simulink model "MOBATSim"  (R2020b)
settings: Solver=FixedStepAuto  StartTime=0.0  StopTime=Sim_t  FixedStep=0.01  MinStep=0.01  RelTol=1e-2
values from neighbouring files (symbols this model uses):
  Vehicles = evalin('base','Vehicles')    [I2V.m]    (also in VehicleSensors.m)
undefined symbols (not defined in the file or in its folder): Sim_Ts
libraries: simulink x50, robotalgslib x10, drivingvehiclecontroller x10, mpcadaslib x10, pid_lib x10
(part 5 of 7)

== system MOBATSim/Vehicle Model 5/Longitudinal and Lateral Controllers/Longitudinal Speed Control/Reference Acceleration Generation ==
  Driving Mode : Inport
  Speed Error : Inport  Port=2
  Actual Speed : Inport  Port=3
  Emergency Brake : Constant  Value=Vehicles(Vehicle_id).dynamics.minDeceleration
  Multiport Switch3 : MultiPortSwitch  Inputs=4
  Saturation Dynamic : simulink/Discontinuities/Saturation Dynamic  OutMin=[]  OutMax=[]  OutDataTypeStr=Inherit: Same as second input  OutDataType=fixdt(1, 16)  OutScaling=2^-10  DoSatur=off
  Simple Gear Logic : MATLAB Function  TreatAsAtomicUnit=on
  Reference Acceleration Command : Outport  VectorParamsAs1DForOutWhenUnconnected=off
  wires:
  Driving Mode/1 -> Multiport Switch3/1
  Speed Error/1 -> Saturation Dynamic/2
  Emergency Brake/1 -> Saturation Dynamic/3, Multiport Switch3/4
  Saturation Dynamic/1 -> Multiport Switch3/5, Multiport Switch3/2, Multiport Switch3/3
  Actual Speed/1 -> Simple Gear Logic/1(speed)
  Multiport Switch3/1 -> Reference Acceleration Command/1
  Simple Gear Logic/1(maxAcc) -> Saturation Dynamic/1

== system MOBATSim/Vehicle Model 5/Longitudinal and Lateral Controllers/Longitudinal Speed Control/Reference speed according to the driving mode ==
  Driving Mode : Inport
  1 : Inport  Port=2
  2 : Inport  Port=3
  4 : Inport  Port=4
  Constant1 : Constant  Value=0
  Max Speed : Saturate  UpperLimit=Vehicles(Vehicle_id).dynamics.maxSpeed  LowerLimit=-100
  Multiport Switch : MultiPortSwitch  Inputs=4
  Reference Speed : Outport
  wires:
  Constant1/1 -> Multiport Switch/4
  Multiport Switch/1 -> Max Speed/1
  Driving Mode/1 -> Multiport Switch/1
  2/1 -> Multiport Switch/3
  1/1 -> Multiport Switch/2
  Max Speed/1 -> Reference Speed/1
  4/1 -> Multiport Switch/5

== system MOBATSim/Vehicle Model 6/Longitudinal and Lateral Controllers/Lateral Motion Control/Pure Pursuit ==
  pose : Inport
  speed : Inport  Port=2
  changeLane : Inport  Port=3
  MATLAB System : MATLABSystem  System=PurePursuit_WPGenerator  Vehicle_id=Vehicle_id  SimulateUsing=Interpreted execution
      mask Type: PurePursuit_WPGenerator
      mask Display:
      | image('MOBATSIM-Icon-Set_9- PurePursuit WP Generator.png');
      | port_label('input',1,'pose');
      | port_label('input',2,'speed');
      | port_label('input',3,'changeLane');
      | port_label('output',1,'nextWPs');
  Pure Pursuit : robotalgslib/Pure Pursuit  DesiredLinearVelocity=Vehicles(Vehicle_id).dynamics.maxSpeed  MaxAngularVelocity=1  LookaheadDistance=6  TargetDirPort=on  SimulateUsing=Code generation
  Terminator : Terminator
  Terminator1 : Terminator
  Wheel Steering Angle Formulation : Subsystem
  SteerCmd : Outport
  wires:
  MATLAB System/1 -> Pure Pursuit/2
  pose/1 -> Pure Pursuit/1, MATLAB System/1
  speed/1 -> MATLAB System/2
  changeLane/1 -> MATLAB System/3
  Pure Pursuit/3 -> Wheel Steering Angle Formulation/1(alpha)
  Pure Pursuit/1 -> Terminator/1
  Pure Pursuit/2 -> Terminator1/1
  Wheel Steering Angle Formulation/1(referenceYawAngle) -> SteerCmd/1

== system MOBATSim/Vehicle Model 6/Longitudinal and Lateral Controllers/Lateral Motion Control/Stanley ==
  pose : Inport
  speed : Inport  Port=2
  changeLane : Inport  Port=3
  Constant5 : Constant
  Deg to Rad : Gain  Gain=pi/180
  Lateral Controller Stanley : drivingvehiclecontroller/Lateral Controller Stanley  ModelType=Kinematic bicycle model  PositionGainF=2.5  PositionGainR=2.5  YawRateGain=0.2  DelayGain=0.2  VehicleMass=1575  Lf=1.2  Lr=1.6  TireStiffness=19000  Wheelbase=3  MaxSteeringAngle=35
      settings: SourceProductBaseCode=DR
  Stanley Reference Pose Generator : MATLABSystem  System=Stanley_RefPoseGenerator  Vehicle_id=Vehicle_id  SimulateUsing=Interpreted execution
      mask Type: Stanley_RefPoseGenerator
      mask Display:
      | image('MOBATSIM-Icon-Set_10- Stanley.png');
      | port_label('input',1,'pose');
      | port_label('input',2,'speed');
      | port_label('input',3,'changeLane');
      | port_label('output',1,'poseOut');
      | port_label('output',2,'referencePose');
  SteerCmd : Outport
  wires:
  Constant5/1 -> Lateral Controller Stanley/4
  Lateral Controller Stanley/1 -> Deg to Rad/1
  changeLane/1 -> Stanley Reference Pose Generator/3
  Stanley Reference Pose Generator/1 -> Lateral Controller Stanley/2
  Stanley Reference Pose Generator/2 -> Lateral Controller Stanley/1
  pose/1 -> Stanley Reference Pose Generator/1
  speed/1 -> Lateral Controller Stanley/3, Stanley Reference Pose Generator/2
  Deg to Rad/1 -> SteerCmd/1

== system MOBATSim/Vehicle Model 6/Longitudinal and Lateral Controllers/Longitudinal Speed Control/Distance to Stop Controller1 ==
  Distance to Stop : Inport
  Compare To Constant : simulink/Logic and Bit Operations/Compare To Constant  relop=>=  const=10  OutDataTypeStr=uint8
  Gain : Gain  Gain=0.08
  Product : Product
  ref speed : Outport  VectorParamsAs1DForOutWhenUnconnected=off
  wires:
  Distance to Stop/1 -> Compare To Constant/1, Gain/1
  Gain/1 -> Product/1
  Compare To Constant/1 -> Product/2
  Product/1 -> ref speed/1

== system MOBATSim/Vehicle Model 6/Longitudinal and Lateral Controllers/Longitudinal Speed Control/Longitudinal Distance Control ==
  note: 1) Add Subsystem or Model blocks as valid variant choices.
      | 2) You cannot connect blocks at this level. At simulation, connectivity is automatically
      | determined, based on the active variant and port name matching.
  Relative distance : Inport
  Lead Speed : Inport  Port=2
  Ego Speed : Inport  Port=3
  MPC-based : Subsystem  VariantControl=MPC-based
  PID-based : Subsystem  VariantControl=PID-based
  Reference Speed : Outport

== system MOBATSim/Vehicle Model 6/Longitudinal and Lateral Controllers/Longitudinal Speed Control/Reference Acceleration Generation ==
  Driving Mode : Inport
  Speed Error : Inport  Port=2
  Actual Speed : Inport  Port=3
  Emergency Brake : Constant  Value=Vehicles(Vehicle_id).dynamics.minDeceleration
  Multiport Switch3 : MultiPortSwitch  Inputs=4
  Saturation Dynamic : simulink/Discontinuities/Saturation Dynamic  OutMin=[]  OutMax=[]  OutDataTypeStr=Inherit: Same as second input  OutDataType=fixdt(1, 16)  OutScaling=2^-10  DoSatur=off
  Simple Gear Logic : MATLAB Function  TreatAsAtomicUnit=on
  Reference Acceleration Command : Outport  VectorParamsAs1DForOutWhenUnconnected=off
  wires:
  Driving Mode/1 -> Multiport Switch3/1
  Speed Error/1 -> Saturation Dynamic/2
  Emergency Brake/1 -> Saturation Dynamic/3, Multiport Switch3/4
  Saturation Dynamic/1 -> Multiport Switch3/5, Multiport Switch3/2, Multiport Switch3/3
  Actual Speed/1 -> Simple Gear Logic/1(speed)
  Multiport Switch3/1 -> Reference Acceleration Command/1
  Simple Gear Logic/1(maxAcc) -> Saturation Dynamic/1

== system MOBATSim/Vehicle Model 6/Longitudinal and Lateral Controllers/Longitudinal Speed Control/Reference speed according to the driving mode ==
  Driving Mode : Inport
  1 : Inport  Port=2
  2 : Inport  Port=3
  4 : Inport  Port=4
  Constant1 : Constant  Value=0
  Max Speed : Saturate  UpperLimit=Vehicles(Vehicle_id).dynamics.maxSpeed  LowerLimit=-100
  Multiport Switch : MultiPortSwitch  Inputs=4
  Reference Speed : Outport
  wires:
  Constant1/1 -> Multiport Switch/4
  Multiport Switch/1 -> Max Speed/1
  Driving Mode/1 -> Multiport Switch/1
  2/1 -> Multiport Switch/3
  1/1 -> Multiport Switch/2
  Max Speed/1 -> Reference Speed/1
  4/1 -> Multiport Switch/5

== system MOBATSim/Vehicle Model 7/Longitudinal and Lateral Controllers/Lateral Motion Control/Pure Pursuit ==
  pose : Inport
  speed : Inport  Port=2
  changeLane : Inport  Port=3
  MATLAB System : MATLABSystem  System=PurePursuit_WPGenerator  Vehicle_id=Vehicle_id  SimulateUsing=Interpreted execution
      mask Type: PurePursuit_WPGenerator
      mask Display:
      | image('MOBATSIM-Icon-Set_9- PurePursuit WP Generator.png');
      | port_label('input',1,'pose');
      | port_label('input',2,'speed');
      | port_label('input',3,'changeLane');
      | port_label('output',1,'nextWPs');
  Pure Pursuit : robotalgslib/Pure Pursuit  DesiredLinearVelocity=Vehicles(Vehicle_id).dynamics.maxSpeed  MaxAngularVelocity=1  LookaheadDistance=6  TargetDirPort=on  SimulateUsing=Code generation
  Terminator : Terminator
  Terminator1 : Terminator
  Wheel Steering Angle Formulation : Subsystem
  SteerCmd : Outport
  wires:
  MATLAB System/1 -> Pure Pursuit/2
  pose/1 -> Pure Pursuit/1, MATLAB System/1
  speed/1 -> MATLAB System/2
  changeLane/1 -> MATLAB System/3
  Pure Pursuit/3 -> Wheel Steering Angle Formulation/1(alpha)
  Pure Pursuit/1 -> Terminator/1
  Pure Pursuit/2 -> Terminator1/1
  Wheel Steering Angle Formulation/1(referenceYawAngle) -> SteerCmd/1

== system MOBATSim/Vehicle Model 7/Longitudinal and Lateral Controllers/Lateral Motion Control/Stanley ==
  pose : Inport
  speed : Inport  Port=2
  changeLane : Inport  Port=3
  Constant5 : Constant
  Deg to Rad : Gain  Gain=pi/180
  Lateral Controller Stanley : drivingvehiclecontroller/Lateral Controller Stanley  ModelType=Kinematic bicycle model  PositionGainF=2.5  PositionGainR=2.5  YawRateGain=0.2  DelayGain=0.2  VehicleMass=1575  Lf=1.2  Lr=1.6  TireStiffness=19000  Wheelbase=3  MaxSteeringAngle=35
      settings: SourceProductBaseCode=DR
  Stanley Reference Pose Generator : MATLABSystem  System=Stanley_RefPoseGenerator  Vehicle_id=Vehicle_id  SimulateUsing=Interpreted execution
      mask Type: Stanley_RefPoseGenerator
      mask Display:
      | image('MOBATSIM-Icon-Set_10- Stanley.png');
      | port_label('input',1,'pose');
      | port_label('input',2,'speed');
      | port_label('input',3,'changeLane');
      | port_label('output',1,'poseOut');
      | port_label('output',2,'referencePose');
  SteerCmd : Outport
  wires:
  Constant5/1 -> Lateral Controller Stanley/4
  Lateral Controller Stanley/1 -> Deg to Rad/1
  changeLane/1 -> Stanley Reference Pose Generator/3
  Stanley Reference Pose Generator/1 -> Lateral Controller Stanley/2
  Stanley Reference Pose Generator/2 -> Lateral Controller Stanley/1
  pose/1 -> Stanley Reference Pose Generator/1
  speed/1 -> Lateral Controller Stanley/3, Stanley Reference Pose Generator/2
  Deg to Rad/1 -> SteerCmd/1

== system MOBATSim/Vehicle Model 7/Longitudinal and Lateral Controllers/Longitudinal Speed Control/Distance to Stop Controller1 ==
  Distance to Stop : Inport
  Compare To Constant : simulink/Logic and Bit Operations/Compare To Constant  relop=>=  const=10  OutDataTypeStr=uint8
  Gain : Gain  Gain=0.08
  Product : Product
  ref speed : Outport  VectorParamsAs1DForOutWhenUnconnected=off
  wires:
  Distance to Stop/1 -> Compare To Constant/1, Gain/1
  Gain/1 -> Product/1
  Compare To Constant/1 -> Product/2
  Product/1 -> ref speed/1

== system MOBATSim/Vehicle Model 7/Longitudinal and Lateral Controllers/Longitudinal Speed Control/Longitudinal Distance Control ==
  note: 1) Add Subsystem or Model blocks as valid variant choices.
      | 2) You cannot connect blocks at this level. At simulation, connectivity is automatically
      | determined, based on the active variant and port name matching.
  Relative distance : Inport
  Lead Speed : Inport  Port=2
  Ego Speed : Inport  Port=3
  MPC-based : Subsystem  VariantControl=MPC-based
  PID-based : Subsystem  VariantControl=PID-based
  Reference Speed : Outport

== system MOBATSim/Vehicle Model 7/Longitudinal and Lateral Controllers/Longitudinal Speed Control/Reference Acceleration Generation ==
  Driving Mode : Inport
  Speed Error : Inport  Port=2
  Actual Speed : Inport  Port=3
  Emergency Brake : Constant  Value=Vehicles(Vehicle_id).dynamics.minDeceleration
  Multiport Switch3 : MultiPortSwitch  Inputs=4
  Saturation Dynamic : simulink/Discontinuities/Saturation Dynamic  OutMin=[]  OutMax=[]  OutDataTypeStr=Inherit: Same as second input  OutDataType=fixdt(1, 16)  OutScaling=2^-10  DoSatur=off
  Simple Gear Logic : MATLAB Function  TreatAsAtomicUnit=on
  Reference Acceleration Command : Outport  VectorParamsAs1DForOutWhenUnconnected=off
  wires:
  Driving Mode/1 -> Multiport Switch3/1
  Speed Error/1 -> Saturation Dynamic/2
  Emergency Brake/1 -> Saturation Dynamic/3, Multiport Switch3/4
  Saturation Dynamic/1 -> Multiport Switch3/5, Multiport Switch3/2, Multiport Switch3/3
  Actual Speed/1 -> Simple Gear Logic/1(speed)
  Multiport Switch3/1 -> Reference Acceleration Command/1
  Simple Gear Logic/1(maxAcc) -> Saturation Dynamic/1

== system MOBATSim/Vehicle Model 7/Longitudinal and Lateral Controllers/Longitudinal Speed Control/Reference speed according to the driving mode ==
  Driving Mode : Inport
  1 : Inport  Port=2
  2 : Inport  Port=3
  4 : Inport  Port=4
  Constant1 : Constant  Value=0
  Max Speed : Saturate  UpperLimit=Vehicles(Vehicle_id).dynamics.maxSpeed  LowerLimit=-100
  Multiport Switch : MultiPortSwitch  Inputs=4
  Reference Speed : Outport
  wires:
  Constant1/1 -> Multiport Switch/4
  Multiport Switch/1 -> Max Speed/1
  Driving Mode/1 -> Multiport Switch/1
  2/1 -> Multiport Switch/3
  1/1 -> Multiport Switch/2
  Max Speed/1 -> Reference Speed/1
  4/1 -> Multiport Switch/5

== system MOBATSim/Vehicle Model 8/Longitudinal and Lateral Controllers/Lateral Motion Control/Pure Pursuit ==
  pose : Inport
  speed : Inport  Port=2
  changeLane : Inport  Port=3
  MATLAB System : MATLABSystem  System=PurePursuit_WPGenerator  Vehicle_id=Vehicle_id  SimulateUsing=Interpreted execution
      mask Type: PurePursuit_WPGenerator
      mask Display:
      | image('MOBATSIM-Icon-Set_9- PurePursuit WP Generator.png');
      | port_label('input',1,'pose');
      | port_label('input',2,'speed');
      | port_label('input',3,'changeLane');
      | port_label('output',1,'nextWPs');
  Pure Pursuit : robotalgslib/Pure Pursuit  DesiredLinearVelocity=Vehicles(Vehicle_id).dynamics.maxSpeed  MaxAngularVelocity=1  LookaheadDistance=6  TargetDirPort=on  SimulateUsing=Code generation
  Terminator : Terminator
  Terminator1 : Terminator
  Wheel Steering Angle Formulation : Subsystem
  SteerCmd : Outport
  wires:
  MATLAB System/1 -> Pure Pursuit/2
  pose/1 -> Pure Pursuit/1, MATLAB System/1
  speed/1 -> MATLAB System/2
  changeLane/1 -> MATLAB System/3
  Pure Pursuit/3 -> Wheel Steering Angle Formulation/1(alpha)
  Pure Pursuit/1 -> Terminator/1
  Pure Pursuit/2 -> Terminator1/1
  Wheel Steering Angle Formulation/1(referenceYawAngle) -> SteerCmd/1

== system MOBATSim/Vehicle Model 8/Longitudinal and Lateral Controllers/Lateral Motion Control/Stanley ==
  pose : Inport
  speed : Inport  Port=2
  changeLane : Inport  Port=3
  Constant5 : Constant
  Deg to Rad : Gain  Gain=pi/180
  Lateral Controller Stanley : drivingvehiclecontroller/Lateral Controller Stanley  ModelType=Kinematic bicycle model  PositionGainF=2.5  PositionGainR=2.5  YawRateGain=0.2  DelayGain=0.2  VehicleMass=1575  Lf=1.2  Lr=1.6  TireStiffness=19000  Wheelbase=3  MaxSteeringAngle=35
      settings: SourceProductBaseCode=DR
  Stanley Reference Pose Generator : MATLABSystem  System=Stanley_RefPoseGenerator  Vehicle_id=Vehicle_id  SimulateUsing=Interpreted execution
      mask Type: Stanley_RefPoseGenerator
      mask Display:
      | image('MOBATSIM-Icon-Set_10- Stanley.png');
      | port_label('input',1,'pose');
      | port_label('input',2,'speed');
      | port_label('input',3,'changeLane');
      | port_label('output',1,'poseOut');
      | port_label('output',2,'referencePose');
  SteerCmd : Outport
  wires:
  Constant5/1 -> Lateral Controller Stanley/4
  Lateral Controller Stanley/1 -> Deg to Rad/1
  changeLane/1 -> Stanley Reference Pose Generator/3
  Stanley Reference Pose Generator/1 -> Lateral Controller Stanley/2
  Stanley Reference Pose Generator/2 -> Lateral Controller Stanley/1
  pose/1 -> Stanley Reference Pose Generator/1
  speed/1 -> Lateral Controller Stanley/3, Stanley Reference Pose Generator/2
  Deg to Rad/1 -> SteerCmd/1

== system MOBATSim/Vehicle Model 8/Longitudinal and Lateral Controllers/Longitudinal Speed Control/Distance to Stop Controller1 ==
  Distance to Stop : Inport
  Compare To Constant : simulink/Logic and Bit Operations/Compare To Constant  relop=>=  const=10  OutDataTypeStr=uint8
  Gain : Gain  Gain=0.08
  Product : Product
  ref speed : Outport  VectorParamsAs1DForOutWhenUnconnected=off
  wires:
  Distance to Stop/1 -> Compare To Constant/1, Gain/1
  Gain/1 -> Product/1
  Compare To Constant/1 -> Product/2
  Product/1 -> ref speed/1

== system MOBATSim/Vehicle Model 8/Longitudinal and Lateral Controllers/Longitudinal Speed Control/Longitudinal Distance Control ==
  note: 1) Add Subsystem or Model blocks as valid variant choices.
      | 2) You cannot connect blocks at this level. At simulation, connectivity is automatically
      | determined, based on the active variant and port name matching.
  Relative distance : Inport
  Lead Speed : Inport  Port=2
  Ego Speed : Inport  Port=3
  MPC-based : Subsystem  VariantControl=MPC-based
  PID-based : Subsystem  VariantControl=PID-based
  Reference Speed : Outport

== system MOBATSim/Vehicle Model 8/Longitudinal and Lateral Controllers/Longitudinal Speed Control/Reference Acceleration Generation ==
  Driving Mode : Inport
  Speed Error : Inport  Port=2
  Actual Speed : Inport  Port=3
  Emergency Brake : Constant  Value=Vehicles(Vehicle_id).dynamics.minDeceleration
  Multiport Switch3 : MultiPortSwitch  Inputs=4
  Saturation Dynamic : simulink/Discontinuities/Saturation Dynamic  OutMin=[]  OutMax=[]  OutDataTypeStr=Inherit: Same as second input  OutDataType=fixdt(1, 16)  OutScaling=2^-10  DoSatur=off
  Simple Gear Logic : MATLAB Function  TreatAsAtomicUnit=on
  Reference Acceleration Command : Outport  VectorParamsAs1DForOutWhenUnconnected=off
  wires:
  Driving Mode/1 -> Multiport Switch3/1
  Speed Error/1 -> Saturation Dynamic/2
  Emergency Brake/1 -> Saturation Dynamic/3, Multiport Switch3/4
  Saturation Dynamic/1 -> Multiport Switch3/5, Multiport Switch3/2, Multiport Switch3/3
  Actual Speed/1 -> Simple Gear Logic/1(speed)
  Multiport Switch3/1 -> Reference Acceleration Command/1
  Simple Gear Logic/1(maxAcc) -> Saturation Dynamic/1

== system MOBATSim/Vehicle Model 8/Longitudinal and Lateral Controllers/Longitudinal Speed Control/Reference speed according to the driving mode ==
  Driving Mode : Inport
  1 : Inport  Port=2
  2 : Inport  Port=3
  4 : Inport  Port=4
  Constant1 : Constant  Value=0
  Max Speed : Saturate  UpperLimit=Vehicles(Vehicle_id).dynamics.maxSpeed  LowerLimit=-100
  Multiport Switch : MultiPortSwitch  Inputs=4
  Reference Speed : Outport
  wires:
  Constant1/1 -> Multiport Switch/4
  Multiport Switch/1 -> Max Speed/1
  Driving Mode/1 -> Multiport Switch/1
  2/1 -> Multiport Switch/3
  1/1 -> Multiport Switch/2
  Max Speed/1 -> Reference Speed/1
  4/1 -> Multiport Switch/5

== system MOBATSim/Vehicle Model 9/Longitudinal and Lateral Controllers/Lateral Motion Control/Pure Pursuit ==
  pose : Inport
  speed : Inport  Port=2
  changeLane : Inport  Port=3
  MATLAB System : MATLABSystem  System=PurePursuit_WPGenerator  Vehicle_id=Vehicle_id  SimulateUsing=Interpreted execution
      mask Type: PurePursuit_WPGenerator
      mask Display:
      | image('MOBATSIM-Icon-Set_9- PurePursuit WP Generator.png');
      | port_label('input',1,'pose');
      | port_label('input',2,'speed');
      | port_label('input',3,'changeLane');
      | port_label('output',1,'nextWPs');
  Pure Pursuit : robotalgslib/Pure Pursuit  DesiredLinearVelocity=Vehicles(Vehicle_id).dynamics.maxSpeed  MaxAngularVelocity=1  LookaheadDistance=6  TargetDirPort=on  SimulateUsing=Code generation
  Terminator : Terminator
  Terminator1 : Terminator
  Wheel Steering Angle Formulation : Subsystem
  SteerCmd : Outport
  wires:
  MATLAB System/1 -> Pure Pursuit/2
  pose/1 -> Pure Pursuit/1, MATLAB System/1
  speed/1 -> MATLAB System/2
  changeLane/1 -> MATLAB System/3
  Pure Pursuit/3 -> Wheel Steering Angle Formulation/1(alpha)
  Pure Pursuit/1 -> Terminator/1
  Pure Pursuit/2 -> Terminator1/1
  Wheel Steering Angle Formulation/1(referenceYawAngle) -> SteerCmd/1

== system MOBATSim/Vehicle Model 9/Longitudinal and Lateral Controllers/Lateral Motion Control/Stanley ==
  pose : Inport
  speed : Inport  Port=2
  changeLane : Inport  Port=3
  Constant5 : Constant
  Deg to Rad : Gain  Gain=pi/180
  Lateral Controller Stanley : drivingvehiclecontroller/Lateral Controller Stanley  ModelType=Kinematic bicycle model  PositionGainF=2.5  PositionGainR=2.5  YawRateGain=0.2  DelayGain=0.2  VehicleMass=1575  Lf=1.2  Lr=1.6  TireStiffness=19000  Wheelbase=3  MaxSteeringAngle=35
      settings: SourceProductBaseCode=DR
  Stanley Reference Pose Generator : MATLABSystem  System=Stanley_RefPoseGenerator  Vehicle_id=Vehicle_id  SimulateUsing=Interpreted execution
      mask Type: Stanley_RefPoseGenerator
      mask Display:
      | image('MOBATSIM-Icon-Set_10- Stanley.png');
      | port_label('input',1,'pose');
      | port_label('input',2,'speed');
      | port_label('input',3,'changeLane');
      | port_label('output',1,'poseOut');
      | port_label('output',2,'referencePose');
  SteerCmd : Outport
  wires:
  Constant5/1 -> Lateral Controller Stanley/4
  Lateral Controller Stanley/1 -> Deg to Rad/1
  changeLane/1 -> Stanley Reference Pose Generator/3
  Stanley Reference Pose Generator/1 -> Lateral Controller Stanley/2
  Stanley Reference Pose Generator/2 -> Lateral Controller Stanley/1
  pose/1 -> Stanley Reference Pose Generator/1
  speed/1 -> Lateral Controller Stanley/3, Stanley Reference Pose Generator/2
  Deg to Rad/1 -> SteerCmd/1

== system MOBATSim/Vehicle Model 9/Longitudinal and Lateral Controllers/Longitudinal Speed Control/Distance to Stop Controller1 ==
  Distance to Stop : Inport
  Compare To Constant : simulink/Logic and Bit Operations/Compare To Constant  relop=>=  const=10  OutDataTypeStr=uint8
  Gain : Gain  Gain=0.08
  Product : Product
  ref speed : Outport  VectorParamsAs1DForOutWhenUnconnected=off
  wires:
  Distance to Stop/1 -> Compare To Constant/1, Gain/1
  Gain/1 -> Product/1
  Compare To Constant/1 -> Product/2
  Product/1 -> ref speed/1

== system MOBATSim/Vehicle Model 9/Longitudinal and Lateral Controllers/Longitudinal Speed Control/Longitudinal Distance Control ==
  note: 1) Add Subsystem or Model blocks as valid variant choices.
      | 2) You cannot connect blocks at this level. At simulation, connectivity is automatically
      | determined, based on the active variant and port name matching.
  Relative distance : Inport
  Lead Speed : Inport  Port=2
  Ego Speed : Inport  Port=3
  MPC-based : Subsystem  VariantControl=MPC-based
  PID-based : Subsystem  VariantControl=PID-based
  Reference Speed : Outport

== system MOBATSim/Vehicle Model 9/Longitudinal and Lateral Controllers/Longitudinal Speed Control/Reference Acceleration Generation ==
  Driving Mode : Inport
  Speed Error : Inport  Port=2
  Actual Speed : Inport  Port=3
  Emergency Brake : Constant  Value=Vehicles(Vehicle_id).dynamics.minDeceleration
  Multiport Switch3 : MultiPortSwitch  Inputs=4
  Saturation Dynamic : simulink/Discontinuities/Saturation Dynamic  OutMin=[]  OutMax=[]  OutDataTypeStr=Inherit: Same as second input  OutDataType=fixdt(1, 16)  OutScaling=2^-10  DoSatur=off
  Simple Gear Logic : MATLAB Function  TreatAsAtomicUnit=on
  Reference Acceleration Command : Outport  VectorParamsAs1DForOutWhenUnconnected=off
  wires:
  Driving Mode/1 -> Multiport Switch3/1
  Speed Error/1 -> Saturation Dynamic/2
  Emergency Brake/1 -> Saturation Dynamic/3, Multiport Switch3/4
  Saturation Dynamic/1 -> Multiport Switch3/5, Multiport Switch3/2, Multiport Switch3/3
  Actual Speed/1 -> Simple Gear Logic/1(speed)
  Multiport Switch3/1 -> Reference Acceleration Command/1
  Simple Gear Logic/1(maxAcc) -> Saturation Dynamic/1

== system MOBATSim/Vehicle Model 9/Longitudinal and Lateral Controllers/Longitudinal Speed Control/Reference speed according to the driving mode ==
  Driving Mode : Inport
  1 : Inport  Port=2
  2 : Inport  Port=3
  4 : Inport  Port=4
  Constant1 : Constant  Value=0
  Max Speed : Saturate  UpperLimit=Vehicles(Vehicle_id).dynamics.maxSpeed  LowerLimit=-100
  Multiport Switch : MultiPortSwitch  Inputs=4
  Reference Speed : Outport
  wires:
  Constant1/1 -> Multiport Switch/4
  Multiport Switch/1 -> Max Speed/1
  Driving Mode/1 -> Multiport Switch/1
  2/1 -> Multiport Switch/3
  1/1 -> Multiport Switch/2
  Max Speed/1 -> Reference Speed/1
  4/1 -> Multiport Switch/5

== system MOBATSim/Vehicle Model 1/Longitudinal and Lateral Controllers/Lateral Motion Control/Pure Pursuit/Wheel Steering Angle Formulation ==
  note: $\delta(t)=tan^{-1} \left( \frac{2\ L\ sin(\alpha)}{l_{d}} \right)$
  alpha : Inport
  Atan : Trigonometry  Operator=atan
  Divide : Product  Inputs=*/
  Gain : Gain  Gain=2
  One over Look Ahead Distance : Constant  Value=6
  Product : Product
  Sine Wave : Sin  TimeSource=Use external signal  SampleTime=0
  Wheel Base : Constant  Value=3
  referenceYawAngle : Outport
  wires:
  Wheel Base/1 -> Gain/1
  Gain/1 -> Product/1
  alpha/1 -> Sine Wave/1
  Sine Wave/1 -> Product/2
  Product/1 -> Divide/1
  One over Look Ahead Distance/1 -> Divide/2
  Divide/1 -> Atan/1
  Atan/1 -> referenceYawAngle/1

== system MOBATSim/Vehicle Model 1/Longitudinal and Lateral Controllers/Longitudinal Speed Control/Longitudinal Distance Control/MPC-based ==
  note: Needs Model Predictive Control Toolbox™ to run
  Relative distance : Inport
  Lead Speed : Inport  Port=2
  Ego Speed : Inport  Port=3
  Adaptive Cruise Control System : mpcadaslib/Adaptive Cruise Control System  EgoModel=tf(1,[1,0])  InitialEgoVelocity=0  DefaultSpacing=Vehicles(Vehicle_id).sensors.safeDistance  MaxVelocity=Vehicles(Vehicle_id).dynamics.maxSpeed  MinAcceleration=-3  amin_ext=off  MaxAcceleration=2  amax_ext=off  Ts=0.4  PredictionHorizon=5  ControllerBehavior=0.620  suboptimal=off  maxiter=10  datatypeopt=double  optmode=off  trackmode=off
  Constant1 : Constant  Value=1.4
  Constant2 : Constant  Value=Vehicles(Vehicle_id).dynamics.maxSpeed
  Integrator1 : Integrator  LimitOutput=on  UpperSaturationLimit=2  LowerSaturationLimit=-3
  Sum : Sum  Inputs=|-+
  Sum4 : Sum  Inputs=|++
  Zero-Order Hold2 : ZeroOrderHold  SampleTime=Sim_Ts
  Reference Speed : Outport  VectorParamsAs1DForOutWhenUnconnected=off
  wires:
  Sum/1 -> Adaptive Cruise Control System/5
  Relative distance/1 -> Adaptive Cruise Control System/4
  Adaptive Cruise Control System/1 -> Integrator1/1
  Integrator1/1 -> Zero-Order Hold2/1
  Sum4/1 -> Reference Speed/1
  Constant1/1 -> Adaptive Cruise Control System/2
  Constant2/1 -> Adaptive Cruise Control System/1
  Lead Speed/1 -> Sum/2
  Ego Speed/1 -> Sum4/2, Adaptive Cruise Control System/3, Sum/1
  Zero-Order Hold2/1 -> Sum4/1

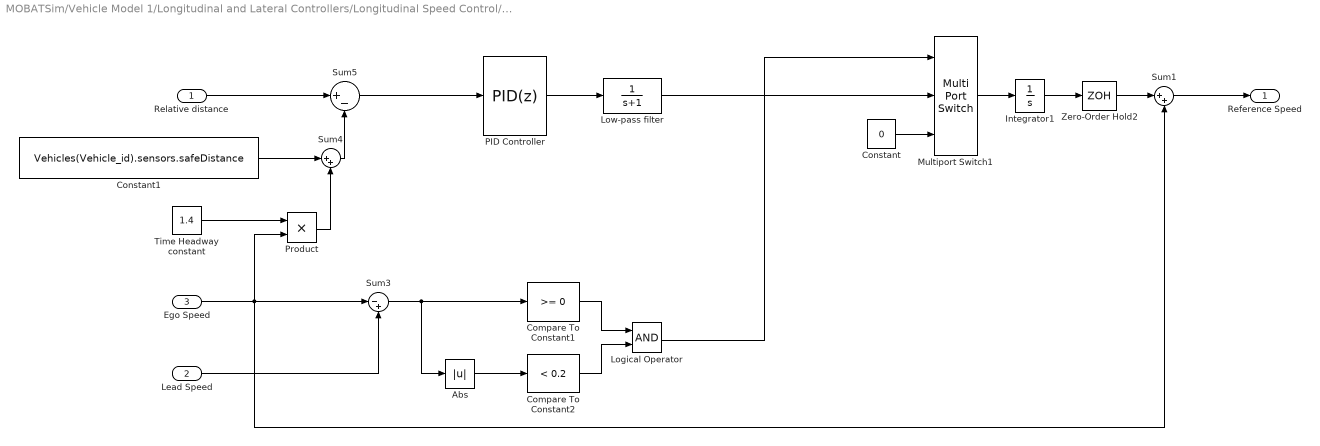
== system MOBATSim/Vehicle Model 1/Longitudinal and Lateral Controllers/Longitudinal Speed Control/Longitudinal Distance Control/PID-based ==
  Relative distance : Inport
  Lead Speed : Inport  Port=2
  Ego Speed : Inport  Port=3
  Abs : Abs
  Compare To Constant1 : simulink/Logic and Bit Operations/Compare To Constant  relop=>=  const=0  OutDataTypeStr=uint8
  Compare To Constant2 : simulink/Logic and Bit Operations/Compare To Constant  relop=<  const=0.2  OutDataTypeStr=uint8
  Constant : Constant  Value=0
  Constant1 : Constant  Value=Vehicles(Vehicle_id).sensors.safeDistance
  Integrator1 : Integrator  LimitOutput=on  UpperSaturationLimit=2  LowerSaturationLimit=-3
  Logical Operator : Logic  AllPortsSameDT=off  OutDataTypeStr=boolean
  Low-pass filter : TransferFcn  Denominator=[1 1]
  Multiport Switch1 : MultiPortSwitch  DataPortOrder=Zero-based contiguous  Inputs=2  zeroidx=on
  PID Controller : pid_lib/PID Controller  Controller=PID  Form=Parallel  TimeDomain=Discrete-time  UseExternalTs=off  SampleTime=0.1  IntegratorMethod=Trapezoidal  FilterMethod=Trapezoidal  ControllerParametersSource=internal  P=1.2  I=0.02  D=0.3  UseFilter=on  N=230  TunerSelectOption=Transfer Function Based (PID Tuner App)  InitialConditionSource=internal  InitialConditionForIntegrator=0  InitialConditionForFilter=0  DifferentiatorICPrevScaledInput=0  ExternalReset=none  TrackingMode=off  Kt=1  LimitOutput=on  SatLimitsSource=internal  UpperSaturationLimit=2  LowerSaturationLimit=-3  LinearizeAsGain=on  AntiWindupMode=back-calculation  Kb=1  POutMin=[]  POutMax=[]  IOutMin=[]  IOutMax=[]  DOutMin=[]  DOutMax=[]  NOutMin=[]  NOutMax=[]  SumOutMin=[]  SumOutMax=[]  SaturationOutMin=[]  SaturationOutMax=[]  PParamMin=[]  PParamMax=[]  IParamMin=[]  IParamMax=[]  DParamMin=[]  DParamMax=[]  NParamMin=[]  NParamMax=[]  KbParamMin=[]  KbParamMax=[]  KtParamMin=[]  KtParamMax=[]  KbOutMin=[]  KbOutMax=[]  KtOutMin=[]  KtOutMax=[]  IntegratorOutMin=[]  IntegratorOutMax=[]  FilterOutMin=[]  FilterOutMax=[]  SumI1OutMin=[]  SumI1OutMax=[]  SumI2OutMin=[]  SumI2OutMax=[]  SumI3OutMin=[]  SumI3OutMax=[]  SumI4OutMin=[]  SumI4OutMax=[]  SumDOutMin=[]  SumDOutMax=[]  DifferentiatorOutMin=[]  DifferentiatorOutMax=[]  FilterDiffOutCoefMin=[]  FilterDiffOutCoefMax=[]  ReciprocalOutMin=[]  ReciprocalOutMax=[]  SumDenOutMin=[]  SumDenOutMax=[]  SumNumOutMin=[]  SumNumOutMax=[]  DivideOutMin=[]  DivideOutMax=[]  UdiffTsProdOutMin=[]  UdiffTsProdOutMax=[]  NTsProdOutMin=[]  NTsProdOutMax=[]  UintegralTsProdOutMin=[]  UintegralTsProdOutMax=[]  UngainTsProdOutMin=[]  UngainTsProdOutMax=[]  IntegratorContinuousStateAttributes=''  IntegratorStateMustResolveToSignalObject=off  IntegratorRTWStateStorageClass=Auto  FilterContinuousStateAttributes=''  FilterStateMustResolveToSignalObject=off  FilterRTWStateStorageClass=Auto  ParallelPVariant=InternalParameters  IdealPVariant=Disabled  IVariant=InternalParameters  DVariant=InternalParameters  IntegratorVariant=Discrete  SatVariant=Enabled  AWVariant=BackCalculation  PCopyVariant=Disabled  TRVariant=Disabled  FdbkBlocksVariant=Feedback  IdealPFdbkVariant=Passthrough  SatFdbkVariant=Enabled  DerivativeFilterVariant=TrapezoidalFilter  NVariant=InternalParameters  NCopyVariant=InternalParameters  FilterICVariant=InternalICsFilter  IntegratorICVariant=InternalICs  ExternalResetVariant=Disabled  TRSumVariant=Passthrough  SumFdbkVariant=Enabled  SumVariant=Sum_PID  TsampFilterVariant=InternalTs  TsampNgainVariant=Passthrough  TsampIntegralVariant=Passthrough  ExternalSaturationOutDataTypeStr=Inherit: Same as second input
  Product : Product
  Sum1 : Sum  Inputs=|++
  Sum3 : Sum  Inputs=|-+
  Sum4 : Sum  Inputs=|++
  Sum5 : Sum  Inputs=|+-
  Time Headway constant : Constant  Value=1.4
  Zero-Order Hold2 : ZeroOrderHold  SampleTime=Sim_Ts
  Reference Speed : Outport  VectorParamsAs1DForOutWhenUnconnected=off
  wires:
  Low-pass filter/1 -> Multiport Switch1/2
  Lead Speed/1 -> Sum3/2
  PID Controller/1 -> Low-pass filter/1
  Time Headway constant/1 -> Product/1
  Constant1/1 -> Sum4/1
  Sum4/1 -> Sum5/2
  Abs/1 -> Compare To Constant2/1
  Logical Operator/1 -> Multiport Switch1/1
  Compare To Constant2/1 -> Logical Operator/2
  Sum5/1 -> PID Controller/1
  Constant/1 -> Multiport Switch1/3
  Product/1 -> Sum4/2
  Relative distance/1 -> Sum5/1
  Sum3/1 -> Abs/1, Compare To Constant1/1
  Compare To Constant1/1 -> Logical Operator/1
  Zero-Order Hold2/1 -> Sum1/1
  Ego Speed/1 -> Product/2, Sum1/2, Sum3/1
  Integrator1/1 -> Zero-Order Hold2/1
  Multiport Switch1/1 -> Integrator1/1
  Sum1/1 -> Reference Speed/1

== system MOBATSim/Vehicle Model 10/Longitudinal and Lateral Controllers/Lateral Motion Control/Pure Pursuit/Wheel Steering Angle Formulation ==
  note: $\delta(t)=tan^{-1} \left( \frac{2\ L\ sin(\alpha)}{l_{d}} \right)$
  alpha : Inport
  Atan : Trigonometry  Operator=atan
  Divide : Product  Inputs=*/
  Gain : Gain  Gain=2
  One over Look Ahead Distance : Constant  Value=6
  Product : Product
  Sine Wave : Sin  TimeSource=Use external signal  SampleTime=0
  Wheel Base : Constant  Value=3
  referenceYawAngle : Outport
  wires:
  Wheel Base/1 -> Gain/1
  Gain/1 -> Product/1
  alpha/1 -> Sine Wave/1
  Sine Wave/1 -> Product/2
  Product/1 -> Divide/1
  One over Look Ahead Distance/1 -> Divide/2
  Divide/1 -> Atan/1
  Atan/1 -> referenceYawAngle/1

== system MOBATSim/Vehicle Model 10/Longitudinal and Lateral Controllers/Longitudinal Speed Control/Longitudinal Distance Control/MPC-based ==
  note: Needs Model Predictive Control Toolbox™ to run
  Relative distance : Inport
  Lead Speed : Inport  Port=2
  Ego Speed : Inport  Port=3
  Adaptive Cruise Control System : mpcadaslib/Adaptive Cruise Control System  EgoModel=tf(1,[1,0])  InitialEgoVelocity=0  DefaultSpacing=Vehicles(Vehicle_id).sensors.safeDistance  MaxVelocity=Vehicles(Vehicle_id).dynamics.maxSpeed  MinAcceleration=-3  amin_ext=off  MaxAcceleration=2  amax_ext=off  Ts=0.4  PredictionHorizon=5  ControllerBehavior=0.620  suboptimal=off  maxiter=10  datatypeopt=double  optmode=off  trackmode=off
  Constant1 : Constant  Value=1.4
  Constant2 : Constant  Value=Vehicles(Vehicle_id).dynamics.maxSpeed
  Integrator1 : Integrator  LimitOutput=on  UpperSaturationLimit=2  LowerSaturationLimit=-3
  Sum : Sum  Inputs=|-+
  Sum4 : Sum  Inputs=|++
  Zero-Order Hold2 : ZeroOrderHold  SampleTime=Sim_Ts
  Reference Speed : Outport  VectorParamsAs1DForOutWhenUnconnected=off
  wires:
  Sum/1 -> Adaptive Cruise Control System/5
  Relative distance/1 -> Adaptive Cruise Control System/4
  Adaptive Cruise Control System/1 -> Integrator1/1
  Integrator1/1 -> Zero-Order Hold2/1
  Sum4/1 -> Reference Speed/1
  Constant1/1 -> Adaptive Cruise Control System/2
  Constant2/1 -> Adaptive Cruise Control System/1
  Lead Speed/1 -> Sum/2
  Ego Speed/1 -> Sum4/2, Adaptive Cruise Control System/3, Sum/1
  Zero-Order Hold2/1 -> Sum4/1

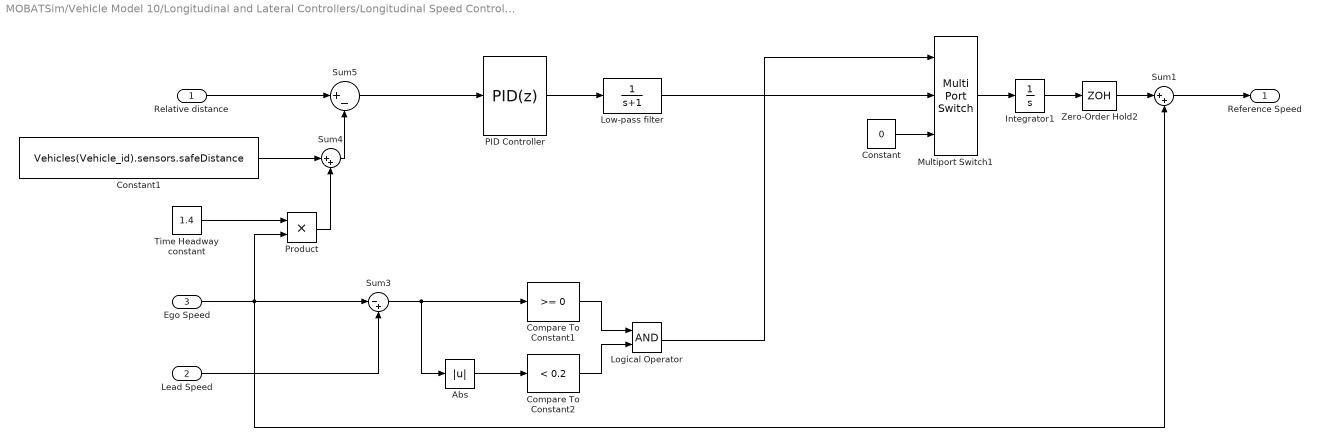
== system MOBATSim/Vehicle Model 10/Longitudinal and Lateral Controllers/Longitudinal Speed Control/Longitudinal Distance Control/PID-based ==
  Relative distance : Inport
  Lead Speed : Inport  Port=2
  Ego Speed : Inport  Port=3
  Abs : Abs
  Compare To Constant1 : simulink/Logic and Bit Operations/Compare To Constant  relop=>=  const=0  OutDataTypeStr=uint8
  Compare To Constant2 : simulink/Logic and Bit Operations/Compare To Constant  relop=<  const=0.2  OutDataTypeStr=uint8
  Constant : Constant  Value=0
  Constant1 : Constant  Value=Vehicles(Vehicle_id).sensors.safeDistance
  Integrator1 : Integrator  LimitOutput=on  UpperSaturationLimit=2  LowerSaturationLimit=-3
  Logical Operator : Logic  AllPortsSameDT=off  OutDataTypeStr=boolean
  Low-pass filter : TransferFcn  Denominator=[1 1]
  Multiport Switch1 : MultiPortSwitch  DataPortOrder=Zero-based contiguous  Inputs=2  zeroidx=on
  PID Controller : pid_lib/PID Controller  Controller=PID  Form=Parallel  TimeDomain=Discrete-time  UseExternalTs=off  SampleTime=0.1  IntegratorMethod=Trapezoidal  FilterMethod=Trapezoidal  ControllerParametersSource=internal  P=1.2  I=0.02  D=0.3  UseFilter=on  N=230  TunerSelectOption=Transfer Function Based (PID Tuner App)  InitialConditionSource=internal  InitialConditionForIntegrator=0  InitialConditionForFilter=0  DifferentiatorICPrevScaledInput=0  ExternalReset=none  TrackingMode=off  Kt=1  LimitOutput=on  SatLimitsSource=internal  UpperSaturationLimit=2  LowerSaturationLimit=-3  LinearizeAsGain=on  AntiWindupMode=back-calculation  Kb=1  POutMin=[]  POutMax=[]  IOutMin=[]  IOutMax=[]  DOutMin=[]  DOutMax=[]  NOutMin=[]  NOutMax=[]  SumOutMin=[]  SumOutMax=[]  SaturationOutMin=[]  SaturationOutMax=[]  PParamMin=[]  PParamMax=[]  IParamMin=[]  IParamMax=[]  DParamMin=[]  DParamMax=[]  NParamMin=[]  NParamMax=[]  KbParamMin=[]  KbParamMax=[]  KtParamMin=[]  KtParamMax=[]  KbOutMin=[]  KbOutMax=[]  KtOutMin=[]  KtOutMax=[]  IntegratorOutMin=[]  IntegratorOutMax=[]  FilterOutMin=[]  FilterOutMax=[]  SumI1OutMin=[]  SumI1OutMax=[]  SumI2OutMin=[]  SumI2OutMax=[]  SumI3OutMin=[]  SumI3OutMax=[]  SumI4OutMin=[]  SumI4OutMax=[]  SumDOutMin=[]  SumDOutMax=[]  DifferentiatorOutMin=[]  DifferentiatorOutMax=[]  FilterDiffOutCoefMin=[]  FilterDiffOutCoefMax=[]  ReciprocalOutMin=[]  ReciprocalOutMax=[]  SumDenOutMin=[]  SumDenOutMax=[]  SumNumOutMin=[]  SumNumOutMax=[]  DivideOutMin=[]  DivideOutMax=[]  UdiffTsProdOutMin=[]  UdiffTsProdOutMax=[]  NTsProdOutMin=[]  NTsProdOutMax=[]  UintegralTsProdOutMin=[]  UintegralTsProdOutMax=[]  UngainTsProdOutMin=[]  UngainTsProdOutMax=[]  IntegratorContinuousStateAttributes=''  IntegratorStateMustResolveToSignalObject=off  IntegratorRTWStateStorageClass=Auto  FilterContinuousStateAttributes=''  FilterStateMustResolveToSignalObject=off  FilterRTWStateStorageClass=Auto  ParallelPVariant=InternalParameters  IdealPVariant=Disabled  IVariant=InternalParameters  DVariant=InternalParameters  IntegratorVariant=Discrete  SatVariant=Enabled  AWVariant=BackCalculation  PCopyVariant=Disabled  TRVariant=Disabled  FdbkBlocksVariant=Feedback  IdealPFdbkVariant=Passthrough  SatFdbkVariant=Enabled  DerivativeFilterVariant=TrapezoidalFilter  NVariant=InternalParameters  NCopyVariant=InternalParameters  FilterICVariant=InternalICsFilter  IntegratorICVariant=InternalICs  ExternalResetVariant=Disabled  TRSumVariant=Passthrough  SumFdbkVariant=Enabled  SumVariant=Sum_PID  TsampFilterVariant=InternalTs  TsampNgainVariant=Passthrough  TsampIntegralVariant=Passthrough  ExternalSaturationOutDataTypeStr=Inherit: Same as second input
  Product : Product
  Sum1 : Sum  Inputs=|++
  Sum3 : Sum  Inputs=|-+
  Sum4 : Sum  Inputs=|++
  Sum5 : Sum  Inputs=|+-
  Time Headway constant : Constant  Value=1.4
  Zero-Order Hold2 : ZeroOrderHold  SampleTime=Sim_Ts
  Reference Speed : Outport  VectorParamsAs1DForOutWhenUnconnected=off
  wires:
  Low-pass filter/1 -> Multiport Switch1/2
  Lead Speed/1 -> Sum3/2
  PID Controller/1 -> Low-pass filter/1
  Time Headway constant/1 -> Product/1
  Constant1/1 -> Sum4/1
  Sum4/1 -> Sum5/2
  Abs/1 -> Compare To Constant2/1
  Logical Operator/1 -> Multiport Switch1/1
  Compare To Constant2/1 -> Logical Operator/2
  Sum5/1 -> PID Controller/1
  Constant/1 -> Multiport Switch1/3
  Product/1 -> Sum4/2
  Relative distance/1 -> Sum5/1
  Sum3/1 -> Abs/1, Compare To Constant1/1
  Compare To Constant1/1 -> Logical Operator/1
  Zero-Order Hold2/1 -> Sum1/1
  Ego Speed/1 -> Product/2, Sum1/2, Sum3/1
  Integrator1/1 -> Zero-Order Hold2/1
  Multiport Switch1/1 -> Integrator1/1
  Sum1/1 -> Reference Speed/1

== system MOBATSim/Vehicle Model 2/Longitudinal and Lateral Controllers/Lateral Motion Control/Pure Pursuit/Target direction to steering angle command ==
  note: $arctan \left( \frac{2\ L_{width}\ sin(\alpha_{dir})}{l_{d}} \right) = \delta(t)$
  alpha : Inport
  2*Wheel Base/Look ahead dist : Constant  Value=2*4/6
  Atan : Trigonometry  Operator=atan
  Product : Product
  Sin : Trigonometry
  Ref Steering Angle : Outport
  wires:
  2*Wheel Base/Look ahead dist/1 -> Product/1
  alpha/1 -> Sin/1
  Sin/1 -> Product/2
  Product/1 -> Atan/1
  Atan/1 -> Ref Steering Angle/1

== system MOBATSim/Vehicle Model 2/Longitudinal and Lateral Controllers/Longitudinal Speed Control/Longitudinal Distance Control/MPC-based ==
  note: Needs Model Predictive Control Toolbox™ to run
  Relative distance : Inport
  Lead Speed : Inport  Port=2
  Ego Speed : Inport  Port=3
  Adaptive Cruise Control System : mpcadaslib/Adaptive Cruise Control System  EgoModel=tf(1,[1,0])  InitialEgoVelocity=0  DefaultSpacing=Vehicles(Vehicle_id).sensors.safeDistance  MaxVelocity=Vehicles(Vehicle_id).dynamics.maxSpeed  MinAcceleration=-3  amin_ext=off  MaxAcceleration=2  amax_ext=off  Ts=0.4  PredictionHorizon=5  ControllerBehavior=0.620  suboptimal=off  maxiter=10  datatypeopt=double  optmode=off  trackmode=off
  Constant1 : Constant  Value=1.4
  Constant2 : Constant  Value=Vehicles(Vehicle_id).dynamics.maxSpeed
  Integrator1 : Integrator  LimitOutput=on  UpperSaturationLimit=2  LowerSaturationLimit=-3
  Sum : Sum  Inputs=|-+
  Sum4 : Sum  Inputs=|++
  Zero-Order Hold2 : ZeroOrderHold  SampleTime=Sim_Ts
  Reference Speed : Outport  VectorParamsAs1DForOutWhenUnconnected=off
  wires:
  Sum/1 -> Adaptive Cruise Control System/5
  Relative distance/1 -> Adaptive Cruise Control System/4
  Adaptive Cruise Control System/1 -> Integrator1/1
  Integrator1/1 -> Zero-Order Hold2/1
  Sum4/1 -> Reference Speed/1
  Constant1/1 -> Adaptive Cruise Control System/2
  Constant2/1 -> Adaptive Cruise Control System/1
  Lead Speed/1 -> Sum/2
  Ego Speed/1 -> Sum4/2, Adaptive Cruise Control System/3, Sum/1
  Zero-Order Hold2/1 -> Sum4/1

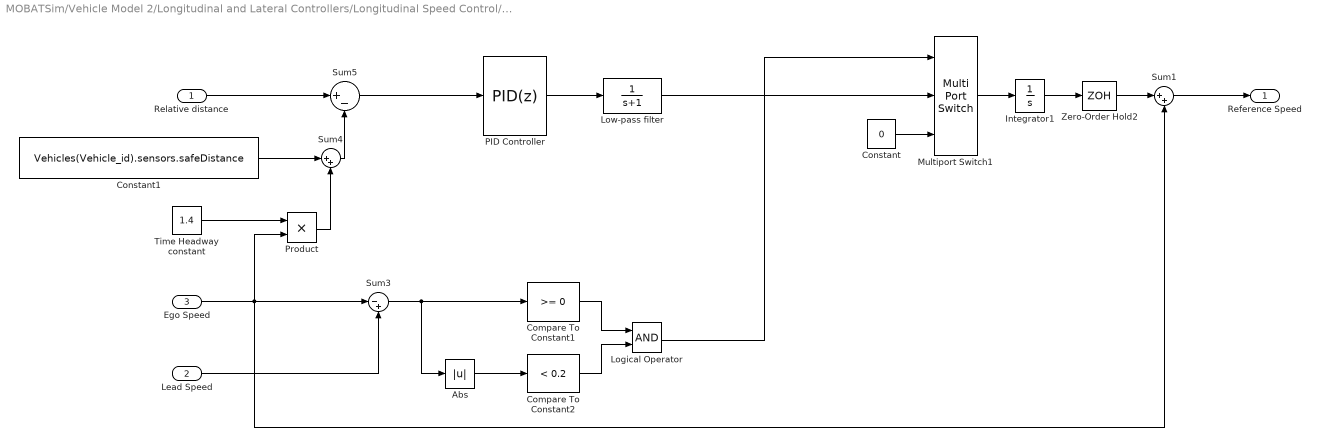
== system MOBATSim/Vehicle Model 2/Longitudinal and Lateral Controllers/Longitudinal Speed Control/Longitudinal Distance Control/PID-based ==
  Relative distance : Inport
  Lead Speed : Inport  Port=2
  Ego Speed : Inport  Port=3
  Abs : Abs
  Compare To Constant1 : simulink/Logic and Bit Operations/Compare To Constant  relop=>=  const=0  OutDataTypeStr=uint8
  Compare To Constant2 : simulink/Logic and Bit Operations/Compare To Constant  relop=<  const=0.2  OutDataTypeStr=uint8
  Constant : Constant  Value=0
  Constant1 : Constant  Value=Vehicles(Vehicle_id).sensors.safeDistance
  Integrator1 : Integrator  LimitOutput=on  UpperSaturationLimit=2  LowerSaturationLimit=-3
  Logical Operator : Logic  AllPortsSameDT=off  OutDataTypeStr=boolean
  Low-pass filter : TransferFcn  Denominator=[1 1]
  Multiport Switch1 : MultiPortSwitch  DataPortOrder=Zero-based contiguous  Inputs=2  zeroidx=on
  PID Controller : pid_lib/PID Controller  Controller=PID  Form=Parallel  TimeDomain=Discrete-time  UseExternalTs=off  SampleTime=0.1  IntegratorMethod=Trapezoidal  FilterMethod=Trapezoidal  ControllerParametersSource=internal  P=1.2  I=0.02  D=0.3  UseFilter=on  N=230  TunerSelectOption=Transfer Function Based (PID Tuner App)  InitialConditionSource=internal  InitialConditionForIntegrator=0  InitialConditionForFilter=0  DifferentiatorICPrevScaledInput=0  ExternalReset=none  TrackingMode=off  Kt=1  LimitOutput=on  SatLimitsSource=internal  UpperSaturationLimit=2  LowerSaturationLimit=-3  LinearizeAsGain=on  AntiWindupMode=back-calculation  Kb=1  POutMin=[]  POutMax=[]  IOutMin=[]  IOutMax=[]  DOutMin=[]  DOutMax=[]  NOutMin=[]  NOutMax=[]  SumOutMin=[]  SumOutMax=[]  SaturationOutMin=[]  SaturationOutMax=[]  PParamMin=[]  PParamMax=[]  IParamMin=[]  IParamMax=[]  DParamMin=[]  DParamMax=[]  NParamMin=[]  NParamMax=[]  KbParamMin=[]  KbParamMax=[]  KtParamMin=[]  KtParamMax=[]  KbOutMin=[]  KbOutMax=[]  KtOutMin=[]  KtOutMax=[]  IntegratorOutMin=[]  IntegratorOutMax=[]  FilterOutMin=[]  FilterOutMax=[]  SumI1OutMin=[]  SumI1OutMax=[]  SumI2OutMin=[]  SumI2OutMax=[]  SumI3OutMin=[]  SumI3OutMax=[]  SumI4OutMin=[]  SumI4OutMax=[]  SumDOutMin=[]  SumDOutMax=[]  DifferentiatorOutMin=[]  DifferentiatorOutMax=[]  FilterDiffOutCoefMin=[]  FilterDiffOutCoefMax=[]  ReciprocalOutMin=[]  ReciprocalOutMax=[]  SumDenOutMin=[]  SumDenOutMax=[]  SumNumOutMin=[]  SumNumOutMax=[]  DivideOutMin=[]  DivideOutMax=[]  UdiffTsProdOutMin=[]  UdiffTsProdOutMax=[]  NTsProdOutMin=[]  NTsProdOutMax=[]  UintegralTsProdOutMin=[]  UintegralTsProdOutMax=[]  UngainTsProdOutMin=[]  UngainTsProdOutMax=[]  IntegratorContinuousStateAttributes=''  IntegratorStateMustResolveToSignalObject=off  IntegratorRTWStateStorageClass=Auto  FilterContinuousStateAttributes=''  FilterStateMustResolveToSignalObject=off  FilterRTWStateStorageClass=Auto  ParallelPVariant=InternalParameters  IdealPVariant=Disabled  IVariant=InternalParameters  DVariant=InternalParameters  IntegratorVariant=Discrete  SatVariant=Enabled  AWVariant=BackCalculation  PCopyVariant=Disabled  TRVariant=Disabled  FdbkBlocksVariant=Feedback  IdealPFdbkVariant=Passthrough  SatFdbkVariant=Enabled  DerivativeFilterVariant=TrapezoidalFilter  NVariant=InternalParameters  NCopyVariant=InternalParameters  FilterICVariant=InternalICsFilter  IntegratorICVariant=InternalICs  ExternalResetVariant=Disabled  TRSumVariant=Passthrough  SumFdbkVariant=Enabled  SumVariant=Sum_PID  TsampFilterVariant=InternalTs  TsampNgainVariant=Passthrough  TsampIntegralVariant=Passthrough  ExternalSaturationOutDataTypeStr=Inherit: Same as second input
  Product : Product
  Sum1 : Sum  Inputs=|++
  Sum3 : Sum  Inputs=|-+
  Sum4 : Sum  Inputs=|++
  Sum5 : Sum  Inputs=|+-
  Time Headway constant : Constant  Value=1.4
  Zero-Order Hold2 : ZeroOrderHold  SampleTime=Sim_Ts
  Reference Speed : Outport  VectorParamsAs1DForOutWhenUnconnected=off
  wires:
  Low-pass filter/1 -> Multiport Switch1/2
  Lead Speed/1 -> Sum3/2
  PID Controller/1 -> Low-pass filter/1
  Time Headway constant/1 -> Product/1
  Constant1/1 -> Sum4/1
  Sum4/1 -> Sum5/2
  Abs/1 -> Compare To Constant2/1
  Logical Operator/1 -> Multiport Switch1/1
  Compare To Constant2/1 -> Logical Operator/2
  Sum5/1 -> PID Controller/1
  Constant/1 -> Multiport Switch1/3
  Product/1 -> Sum4/2
  Relative distance/1 -> Sum5/1
  Sum3/1 -> Abs/1, Compare To Constant1/1
  Compare To Constant1/1 -> Logical Operator/1
  Zero-Order Hold2/1 -> Sum1/1
  Ego Speed/1 -> Product/2, Sum1/2, Sum3/1
  Integrator1/1 -> Zero-Order Hold2/1
  Multiport Switch1/1 -> Integrator1/1
  Sum1/1 -> Reference Speed/1

== system MOBATSim/Vehicle Model 3/Longitudinal and Lateral Controllers/Lateral Motion Control/Pure Pursuit/Wheel Steering Angle Formulation ==
  note: $\delta(t)=tan^{-1} \left( \frac{2\ L\ sin(\alpha)}{l_{d}} \right)$
  alpha : Inport
  Atan : Trigonometry  Operator=atan
  Divide : Product  Inputs=*/
  Gain : Gain  Gain=2
  One over Look Ahead Distance : Constant  Value=6
  Product : Product
  Sine Wave : Sin  TimeSource=Use external signal  SampleTime=0
  Wheel Base : Constant  Value=3
  referenceYawAngle : Outport
  wires:
  Wheel Base/1 -> Gain/1
  Gain/1 -> Product/1
  alpha/1 -> Sine Wave/1
  Sine Wave/1 -> Product/2
  Product/1 -> Divide/1
  One over Look Ahead Distance/1 -> Divide/2
  Divide/1 -> Atan/1
  Atan/1 -> referenceYawAngle/1

== system MOBATSim/Vehicle Model 3/Longitudinal and Lateral Controllers/Longitudinal Speed Control/Longitudinal Distance Control/MPC-based ==
  note: Needs Model Predictive Control Toolbox™ to run
  Relative distance : Inport
  Lead Speed : Inport  Port=2
  Ego Speed : Inport  Port=3
  Adaptive Cruise Control System : mpcadaslib/Adaptive Cruise Control System  EgoModel=tf(1,[1,0])  InitialEgoVelocity=0  DefaultSpacing=Vehicles(Vehicle_id).sensors.safeDistance  MaxVelocity=Vehicles(Vehicle_id).dynamics.maxSpeed  MinAcceleration=-3  amin_ext=off  MaxAcceleration=2  amax_ext=off  Ts=0.4  PredictionHorizon=5  ControllerBehavior=0.620  suboptimal=off  maxiter=10  datatypeopt=double  optmode=off  trackmode=off
  Constant1 : Constant  Value=1.4
  Constant2 : Constant  Value=Vehicles(Vehicle_id).dynamics.maxSpeed
  Integrator1 : Integrator  LimitOutput=on  UpperSaturationLimit=2  LowerSaturationLimit=-3
  Sum : Sum  Inputs=|-+
  Sum4 : Sum  Inputs=|++
  Zero-Order Hold2 : ZeroOrderHold  SampleTime=Sim_Ts
  Reference Speed : Outport  VectorParamsAs1DForOutWhenUnconnected=off
  wires:
  Sum/1 -> Adaptive Cruise Control System/5
  Relative distance/1 -> Adaptive Cruise Control System/4
  Adaptive Cruise Control System/1 -> Integrator1/1
  Integrator1/1 -> Zero-Order Hold2/1
  Sum4/1 -> Reference Speed/1
  Constant1/1 -> Adaptive Cruise Control System/2
  Constant2/1 -> Adaptive Cruise Control System/1
  Lead Speed/1 -> Sum/2
  Ego Speed/1 -> Sum4/2, Adaptive Cruise Control System/3, Sum/1
  Zero-Order Hold2/1 -> Sum4/1
